simulink model "all_pm_0001_0080"  (R2026a)
settings: Solver=FixedStepAuto  StopTime=50  FixedStep=1e-3  EnableMultiTasking=on
settings Model: PacingRate=0.250000  ExtModeTrigDuration=5  Creator=Arun Mistry  LastModifiedBy=harry_31916
settings OptimizationCC: DefaultUnderspecifiedDataType=single
settings HardwareCC: ProdLargestAtomicInteger=Long  ProdLargestAtomicFloat=Double  ProdHWDeviceType=ARM Compatible->ARM Cortex
settings SFSimCC: SimParseCustomCode=off
settings RTWCC: SystemTargetFile=ert.tlc  Toolchain=GNU Tools for ARM Embedded Processors  Description=Embedded Coder
settings ERTTargetCC: DynamicArrayContainerType=coder::array

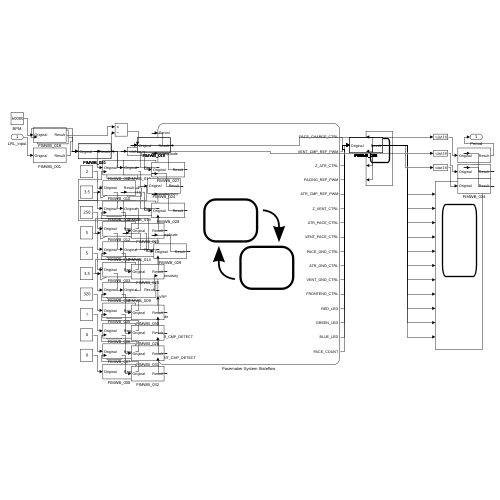
[thumbnail: Simulink's stored preview of the top-level diagram]
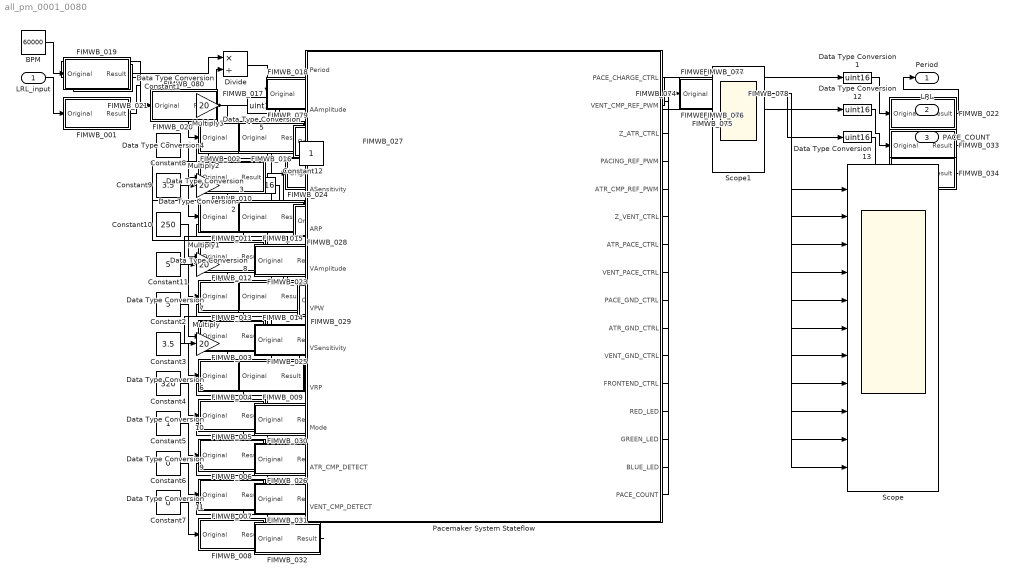
== system all_pm_0001_0080 ==
  LRL_input : Inport  OutDataTypeStr=double
  BPM : Constant  Value=60000
  Constant1 : Constant  Value=5
  Constant10 : Constant  Value=250
  Constant11 : Constant  Value=5
  Constant2 : Constant  Value=5
  Constant3 : Constant  Value=3.5
  Constant4 : Constant  Value=320
  Constant5 : Constant
  Constant6 : Constant  Value=0
  Constant7 : Constant  Value=0
  Constant8 : Constant  Value=2
  Constant9 : Constant  Value=3.5
  Data Type Conversion{,1..8,10,12..13} (12 alike) : DataTypeConversion  OutDataTypeStr=uint16  SaturateOnIntegerOverflow=off  RndMeth=Floor
  Data Type Conversion11 : DataTypeConversion  OutDataTypeStr=boolean  SaturateOnIntegerOverflow=off  RndMeth=Floor
  Data Type Conversion9 : DataTypeConversion  OutDataTypeStr=boolean  SaturateOnIntegerOverflow=off  RndMeth=Floor
  Divide : Product  Inputs=*/
  FIMWB_001 : Subsystem  Tag=fimwb.fault.1
  FIMWB_002 : Subsystem  Tag=fimwb.fault.2
  FIMWB_003 : Subsystem  Tag=fimwb.fault.3
  FIMWB_004 : Subsystem  Tag=fimwb.fault.4
  FIMWB_005 : Subsystem  Tag=fimwb.fault.5
  FIMWB_006 : Subsystem  Tag=fimwb.fault.6
  FIMWB_007 : Subsystem  Tag=fimwb.fault.7
  FIMWB_008 : Subsystem  Tag=fimwb.fault.8
  FIMWB_009 : Subsystem  Tag=fimwb.fault.9
  FIMWB_010 : Subsystem  Tag=fimwb.fault.10
  FIMWB_011 : Subsystem  Tag=fimwb.fault.11
  FIMWB_012 : Subsystem  Tag=fimwb.fault.12
  FIMWB_013 : Subsystem  Tag=fimwb.fault.13
  FIMWB_014 : Subsystem  Tag=fimwb.fault.14
  FIMWB_015 : Subsystem  Tag=fimwb.fault.15
  FIMWB_016 : Subsystem  Tag=fimwb.fault.16
  FIMWB_017 : Subsystem  Tag=fimwb.fault.17
  FIMWB_018 : Subsystem  Tag=fimwb.fault.18
  FIMWB_019 : Subsystem  Tag=fimwb.fault.19
  FIMWB_020 : Subsystem  Tag=fimwb.fault.20
  FIMWB_021 : Subsystem  Tag=fimwb.fault.21
  FIMWB_022 : Subsystem  Tag=fimwb.fault.22
  FIMWB_023 : Subsystem  Tag=fimwb.fault.23
  FIMWB_024 : Subsystem  Tag=fimwb.fault.24
  FIMWB_025 : Subsystem  Tag=fimwb.fault.25
  FIMWB_026 : Subsystem  Tag=fimwb.fault.26
  FIMWB_027 : Subsystem  Tag=fimwb.fault.27
  FIMWB_028 : Subsystem  Tag=fimwb.fault.28
  FIMWB_029 : Subsystem  Tag=fimwb.fault.29
  FIMWB_030 : Subsystem  Tag=fimwb.fault.30
  FIMWB_031 : Subsystem  Tag=fimwb.fault.31
  FIMWB_032 : Subsystem  Tag=fimwb.fault.32
  FIMWB_033 : Subsystem  Tag=fimwb.fault.33
  FIMWB_034 : Subsystem  Tag=fimwb.fault.34
  FIMWB_063 : Subsystem  Tag=fimwb.fault.63
  FIMWB_064 : Subsystem  Tag=fimwb.fault.64
  FIMWB_065 : Subsystem  Tag=fimwb.fault.65
  FIMWB_066 : Subsystem  Tag=fimwb.fault.66
  FIMWB_067 : Subsystem  Tag=fimwb.fault.67
  FIMWB_068 : Subsystem  Tag=fimwb.fault.68
  FIMWB_069 : Subsystem  Tag=fimwb.fault.69
  FIMWB_070 : Subsystem  Tag=fimwb.fault.70
  FIMWB_071 : Subsystem  Tag=fimwb.fault.71
  FIMWB_072 : Subsystem  Tag=fimwb.fault.72
  FIMWB_073 : Subsystem  Tag=fimwb.fault.73
  FIMWB_074 : Subsystem  Tag=fimwb.fault.74
  FIMWB_075 : Subsystem  Tag=fimwb.fault.75
  FIMWB_076 : Subsystem  Tag=fimwb.fault.76
  FIMWB_077 : Subsystem  Tag=fimwb.fault.77
  FIMWB_078 : Subsystem  Tag=fimwb.fault.78
  FIMWB_079 : Subsystem  Tag=fimwb.fault.79
  FIMWB_080 : Subsystem  Tag=fimwb.fault.80
  Multiply{,1..3} (4 alike) : Gain  Gain=20
  Pacemaker System Stateflow : Stateflow chart  TreatAsAtomicUnit=on
  Scope : Scope  NumInputPorts=11
  Scope1 : Scope  NumInputPorts=4
  Period : Outport  OutDataTypeStr=uint16
  LRL : Outport  Port=2  OutDataTypeStr=uint16
  PACE_COUNT : Outport  Port=3
  Constant12 : Constant  IOType=siggen
  wires:
  Divide/1 -> FIMWB_079/1(Original)
  FIMWB_079/1(Result) -> FIMWB_017/1(Original), FIMWB_018/1(Original)
  Data Type Conversion/1 -> FIMWB_080/1(Original)
  FIMWB_080/1(Result) -> FIMWB_020/1(Original), FIMWB_021/1(Original)
  LRL_input/1 -> FIMWB_001/1(Original)
  FIMWB_001/1(Result) -> Data Type Conversion/1
  Constant1/1 -> FIMWB_002/1(Original)
  FIMWB_002/1(Result) -> Multiply3/1
  Constant2/1 -> FIMWB_003/1(Original)
  FIMWB_003/1(Result) -> Data Type Conversion7/1
  Constant3/1 -> FIMWB_004/1(Original)
  FIMWB_004/1(Result) -> Multiply/1
  Constant4/1 -> FIMWB_005/1(Original)
  FIMWB_005/1(Result) -> Data Type Conversion6/1
  Constant5/1 -> FIMWB_006/1(Original)
  FIMWB_006/1(Result) -> Data Type Conversion10/1
  Constant6/1 -> FIMWB_007/1(Original)
  FIMWB_007/1(Result) -> Data Type Conversion9/1
  Constant7/1 -> FIMWB_008/1(Original)
  FIMWB_008/1(Result) -> Data Type Conversion11/1
  Multiply/1 -> FIMWB_009/1(Original)
  FIMWB_009/1(Result) -> Pacemaker System Stateflow/8(VSensitivity)
  Constant8/1 -> FIMWB_010/1(Original)
  FIMWB_010/1(Result) -> Data Type Conversion4/1
  Constant9/1 -> FIMWB_011/1(Original)
  FIMWB_011/1(Result) -> Multiply2/1
  Constant10/1 -> FIMWB_012/1(Original)
  FIMWB_012/1(Result) -> Data Type Conversion2/1
  Constant11/1 -> FIMWB_013/1(Original)
  FIMWB_013/1(Result) -> Multiply1/1
  Multiply1/1 -> FIMWB_014/1(Original)
  FIMWB_014/1(Result) -> Data Type Conversion8/1
  Multiply2/1 -> FIMWB_015/1(Original)
  FIMWB_015/1(Result) -> Data Type Conversion3/1
  Multiply3/1 -> FIMWB_016/1(Original)
  FIMWB_016/1(Result) -> Data Type Conversion5/1
  FIMWB_017/1(Result) -> Data Type Conversion1/1
  FIMWB_018/1(Result) -> Pacemaker System Stateflow/1(Period)
  BPM/1 -> FIMWB_019/1(Original)
  FIMWB_019/1(Result) -> Divide/1
  FIMWB_020/1(Result) -> Divide/2
  FIMWB_021/1(Result) -> Data Type Conversion12/1
  Data Type Conversion1/1 -> FIMWB_022/1(Original)
  FIMWB_022/1(Result) -> Period/1
  Data Type Conversion2/1 -> FIMWB_023/1(Original)
  FIMWB_023/1(Result) -> Pacemaker System Stateflow/5(ARP)
  Data Type Conversion4/1 -> FIMWB_024/1(Original)
  FIMWB_024/1(Result) -> Pacemaker System Stateflow/3(APW)
  Data Type Conversion7/1 -> FIMWB_025/1(Original)
  FIMWB_025/1(Result) -> Pacemaker System Stateflow/7(VPW)
  Data Type Conversion10/1 -> FIMWB_026/1(Original)
  FIMWB_026/1(Result) -> Pacemaker System Stateflow/10(Mode)
  Data Type Conversion5/1 -> FIMWB_027/1(Original)
  FIMWB_027/1(Result) -> Pacemaker System Stateflow/2(AAmplitude)
  Data Type Conversion3/1 -> FIMWB_028/1(Original)
  FIMWB_028/1(Result) -> Pacemaker System Stateflow/4(ASensitivity)
  Data Type Conversion8/1 -> FIMWB_029/1(Original)
  FIMWB_029/1(Result) -> Pacemaker System Stateflow/6(VAmplitude)
  Data Type Conversion6/1 -> FIMWB_030/1(Original)
  FIMWB_030/1(Result) -> Pacemaker System Stateflow/9(VRP)
  Data Type Conversion9/1 -> FIMWB_031/1(Original)
  FIMWB_031/1(Result) -> Pacemaker System Stateflow/11(ATR_CMP_DETECT)
  Data Type Conversion11/1 -> FIMWB_032/1(Original)
  FIMWB_032/1(Result) -> Pacemaker System Stateflow/12(VENT_CMP_DETECT)
  Data Type Conversion12/1 -> FIMWB_033/1(Original)
  FIMWB_033/1(Result) -> LRL/1
  Data Type Conversion13/1 -> FIMWB_034/1(Original)
  FIMWB_034/1(Result) -> PACE_COUNT/1
  Pacemaker System Stateflow/10(ATR_GND_CTRL) -> FIMWB_063/1(Original)
  FIMWB_063/1(Result) -> Scope/6
  Pacemaker System Stateflow/11(VENT_GND_CTRL) -> FIMWB_064/1(Original)
  FIMWB_064/1(Result) -> Scope/7
  Pacemaker System Stateflow/12(FRONTEND_CTRL) -> FIMWB_065/1(Original)
  FIMWB_065/1(Result) -> Scope/8
  Pacemaker System Stateflow/13(RED_LED) -> FIMWB_066/1(Original)
  FIMWB_066/1(Result) -> Scope/9
  Pacemaker System Stateflow/14(GREEN_LED) -> FIMWB_067/1(Original)
  FIMWB_067/1(Result) -> Scope/10
  Pacemaker System Stateflow/15(BLUE_LED) -> FIMWB_068/1(Original)
  FIMWB_068/1(Result) -> Scope/11
  Pacemaker System Stateflow/16(PACE_COUNT) -> FIMWB_069/1(Original)
  FIMWB_069/1(Result) -> Data Type Conversion13/1
  Pacemaker System Stateflow/1(PACE_CHARGE_CTRL) -> FIMWB_070/1(Original)
  FIMWB_070/1(Result) -> Scope1/1
  Pacemaker System Stateflow/2(VENT_CMP_REF_PWM) -> FIMWB_071/1(Original)
  FIMWB_071/1(Result) -> Scope1/2
  Pacemaker System Stateflow/3(Z_ATR_CTRL) -> FIMWB_072/1(Original)
  FIMWB_072/1(Result) -> Scope1/3
  Pacemaker System Stateflow/4(PACING_REF_PWM) -> FIMWB_073/1(Original)
  FIMWB_073/1(Result) -> Scope1/4
  Pacemaker System Stateflow/5(ATR_CMP_REF_PWM) -> FIMWB_074/1(Original)
  FIMWB_074/1(Result) -> Scope/1
  Pacemaker System Stateflow/6(Z_VENT_CTRL) -> FIMWB_075/1(Original)
  FIMWB_075/1(Result) -> Scope/2
  Pacemaker System Stateflow/7(ATR_PACE_CTRL) -> FIMWB_076/1(Original)
  FIMWB_076/1(Result) -> Scope/3
  Pacemaker System Stateflow/8(VENT_PACE_CTRL) -> FIMWB_077/1(Original)
  FIMWB_077/1(Result) -> Scope/4
  Pacemaker System Stateflow/9(PACE_GND_CTRL) -> FIMWB_078/1(Original)
  FIMWB_078/1(Result) -> Scope/5

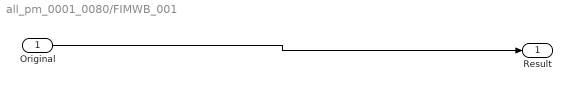
== system all_pm_0001_0080/FIMWB_001 ==
  Original : Inport
  Result : Outport
  wires:
  Original/1 -> Result/1

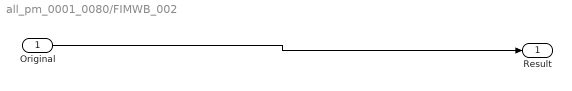
== system all_pm_0001_0080/FIMWB_002 ==
  Original : Inport
  Result : Outport
  wires:
  Original/1 -> Result/1

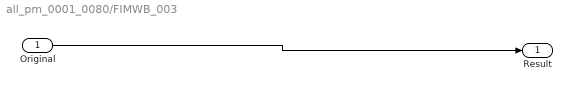
== system all_pm_0001_0080/FIMWB_003 ==
  Original : Inport
  Result : Outport
  wires:
  Original/1 -> Result/1

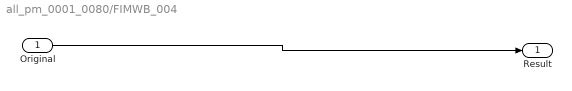
== system all_pm_0001_0080/FIMWB_004 ==
  Original : Inport
  Result : Outport
  wires:
  Original/1 -> Result/1

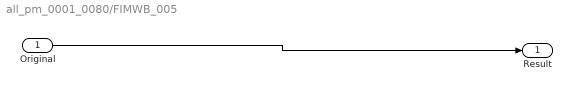
== system all_pm_0001_0080/FIMWB_005 ==
  Original : Inport
  Result : Outport
  wires:
  Original/1 -> Result/1

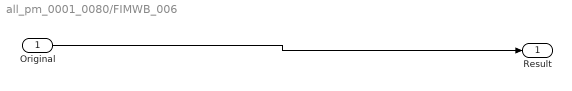
== system all_pm_0001_0080/FIMWB_006 ==
  Original : Inport
  Result : Outport
  wires:
  Original/1 -> Result/1

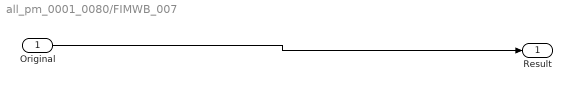
== system all_pm_0001_0080/FIMWB_007 ==
  Original : Inport
  Result : Outport
  wires:
  Original/1 -> Result/1

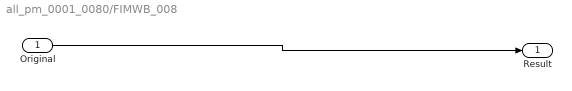
== system all_pm_0001_0080/FIMWB_008 ==
  Original : Inport
  Result : Outport
  wires:
  Original/1 -> Result/1

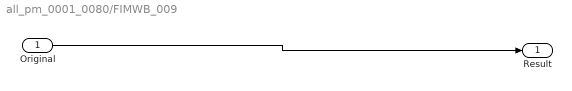
== system all_pm_0001_0080/FIMWB_009 ==
  Original : Inport
  Result : Outport
  wires:
  Original/1 -> Result/1

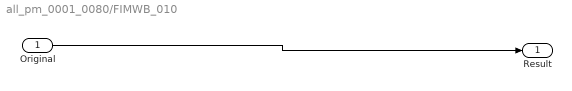
== system all_pm_0001_0080/FIMWB_010 ==
  Original : Inport
  Result : Outport
  wires:
  Original/1 -> Result/1

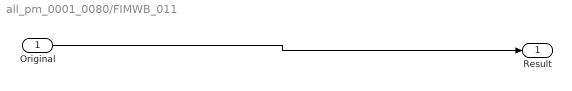
== system all_pm_0001_0080/FIMWB_011 ==
  Original : Inport
  Result : Outport
  wires:
  Original/1 -> Result/1

== system all_pm_0001_0080/FIMWB_012 ==
  Original : Inport
  Result : Outport
  wires:
  Original/1 -> Result/1

== system all_pm_0001_0080/FIMWB_013 ==
  Original : Inport
  Result : Outport
  wires:
  Original/1 -> Result/1

== system all_pm_0001_0080/FIMWB_014 ==
  Original : Inport
  Result : Outport
  wires:
  Original/1 -> Result/1

== system all_pm_0001_0080/FIMWB_015 ==
  Original : Inport
  Result : Outport
  wires:
  Original/1 -> Result/1

== system all_pm_0001_0080/FIMWB_016 ==
  Original : Inport
  Result : Outport
  wires:
  Original/1 -> Result/1

== system all_pm_0001_0080/FIMWB_017 ==
  Original : Inport
  Result : Outport
  wires:
  Original/1 -> Result/1

== system all_pm_0001_0080/FIMWB_018 ==
  Original : Inport
  Result : Outport
  wires:
  Original/1 -> Result/1

== system all_pm_0001_0080/FIMWB_019 ==
  Original : Inport
  Result : Outport
  wires:
  Original/1 -> Result/1

== system all_pm_0001_0080/FIMWB_020 ==
  Original : Inport
  Result : Outport
  wires:
  Original/1 -> Result/1

== system all_pm_0001_0080/FIMWB_021 ==
  Original : Inport
  Result : Outport
  wires:
  Original/1 -> Result/1

== system all_pm_0001_0080/FIMWB_022 ==
  Original : Inport
  Result : Outport
  wires:
  Original/1 -> Result/1

== system all_pm_0001_0080/FIMWB_023 ==
  Original : Inport
  Result : Outport
  wires:
  Original/1 -> Result/1

== system all_pm_0001_0080/FIMWB_024 ==
  Original : Inport
  Result : Outport
  wires:
  Original/1 -> Result/1

== system all_pm_0001_0080/FIMWB_025 ==
  Original : Inport
  Result : Outport
  wires:
  Original/1 -> Result/1

== system all_pm_0001_0080/FIMWB_026 ==
  Original : Inport
  Result : Outport
  wires:
  Original/1 -> Result/1

== system all_pm_0001_0080/FIMWB_027 ==
  Original : Inport
  Result : Outport
  wires:
  Original/1 -> Result/1

== system all_pm_0001_0080/FIMWB_028 ==
  Original : Inport
  Result : Outport
  wires:
  Original/1 -> Result/1

== system all_pm_0001_0080/FIMWB_029 ==
  Original : Inport
  Result : Outport
  wires:
  Original/1 -> Result/1

== system all_pm_0001_0080/FIMWB_030 ==
  Original : Inport
  Result : Outport
  wires:
  Original/1 -> Result/1

== system all_pm_0001_0080/FIMWB_031 ==
  Original : Inport
  Result : Outport
  wires:
  Original/1 -> Result/1

== system all_pm_0001_0080/FIMWB_032 ==
  Original : Inport
  Result : Outport
  wires:
  Original/1 -> Result/1

== system all_pm_0001_0080/FIMWB_033 ==
  Original : Inport
  Result : Outport
  wires:
  Original/1 -> Result/1

== system all_pm_0001_0080/FIMWB_034 ==
  Original : Inport
  Result : Outport
  wires:
  Original/1 -> Result/1

== system all_pm_0001_0080/FIMWB_063 ==
  Original : Inport
  Result : Outport
  wires:
  Original/1 -> Result/1

== system all_pm_0001_0080/FIMWB_064 ==
  Original : Inport
  Result : Outport
  wires:
  Original/1 -> Result/1

== system all_pm_0001_0080/FIMWB_065 ==
  Original : Inport
  Result : Outport
  wires:
  Original/1 -> Result/1

== system all_pm_0001_0080/FIMWB_066 ==
  Original : Inport
  Result : Outport
  wires:
  Original/1 -> Result/1

== system all_pm_0001_0080/FIMWB_067 ==
  Original : Inport
  Result : Outport
  wires:
  Original/1 -> Result/1

== system all_pm_0001_0080/FIMWB_068 ==
  Original : Inport
  Result : Outport
  wires:
  Original/1 -> Result/1

== system all_pm_0001_0080/FIMWB_069 ==
  Original : Inport
  Result : Outport
  wires:
  Original/1 -> Result/1

== system all_pm_0001_0080/FIMWB_070 ==
  Original : Inport
  Result : Outport
  wires:
  Original/1 -> Result/1

== system all_pm_0001_0080/FIMWB_071 ==
  Original : Inport
  Result : Outport
  wires:
  Original/1 -> Result/1

== system all_pm_0001_0080/FIMWB_072 ==
  Original : Inport
  Result : Outport
  wires:
  Original/1 -> Result/1

== system all_pm_0001_0080/FIMWB_073 ==
  Original : Inport
  Result : Outport
  wires:
  Original/1 -> Result/1

== system all_pm_0001_0080/FIMWB_074 ==
  Original : Inport
  Result : Outport
  wires:
  Original/1 -> Result/1

== system all_pm_0001_0080/FIMWB_075 ==
  Original : Inport
  Result : Outport
  wires:
  Original/1 -> Result/1

== system all_pm_0001_0080/FIMWB_076 ==
  Original : Inport
  Result : Outport
  wires:
  Original/1 -> Result/1

== system all_pm_0001_0080/FIMWB_077 ==
  Original : Inport
  Result : Outport
  wires:
  Original/1 -> Result/1

== system all_pm_0001_0080/FIMWB_078 ==
  Original : Inport
  Result : Outport
  wires:
  Original/1 -> Result/1

== system all_pm_0001_0080/FIMWB_079 ==
  Original : Inport
  Result : Outport
  wires:
  Original/1 -> Result/1

== system all_pm_0001_0080/FIMWB_080 ==
  Original : Inport
  Result : Outport
  wires:
  Original/1 -> Result/1

== system all_pm_0001_0080/Pacemaker System Stateflow/FIMWB_035 ==
  Original : Inport
  Result : Outport
  wires:
  Original/1 -> Result/1

== system all_pm_0001_0080/Pacemaker System Stateflow/FIMWB_036 ==
  Original : Inport
  Result : Outport
  wires:
  Original/1 -> Result/1

== system all_pm_0001_0080/Pacemaker System Stateflow/FIMWB_037 ==
  Original : Inport
  Result : Outport
  wires:
  Original/1 -> Result/1

== system all_pm_0001_0080/Pacemaker System Stateflow/FIMWB_038 ==
  Original : Inport
  Result : Outport
  wires:
  Original/1 -> Result/1

== system all_pm_0001_0080/Pacemaker System Stateflow/FIMWB_039 ==
  Original : Inport
  Result : Outport
  wires:
  Original/1 -> Result/1

== system all_pm_0001_0080/Pacemaker System Stateflow/FIMWB_040 ==
  Original : Inport
  Result : Outport
  wires:
  Original/1 -> Result/1

== system all_pm_0001_0080/Pacemaker System Stateflow/FIMWB_041 ==
  Original : Inport
  Result : Outport
  wires:
  Original/1 -> Result/1

== system all_pm_0001_0080/Pacemaker System Stateflow/FIMWB_042 ==
  Original : Inport
  Result : Outport
  wires:
  Original/1 -> Result/1

== system all_pm_0001_0080/Pacemaker System Stateflow/FIMWB_043 ==
  Original : Inport
  Result : Outport
  wires:
  Original/1 -> Result/1

== system all_pm_0001_0080/Pacemaker System Stateflow/FIMWB_044 ==
  Original : Inport
  Result : Outport
  wires:
  Original/1 -> Result/1

== system all_pm_0001_0080/Pacemaker System Stateflow/FIMWB_045 ==
  Original : Inport
  Result : Outport
  wires:
  Original/1 -> Result/1

== system all_pm_0001_0080/Pacemaker System Stateflow/FIMWB_046 ==
  Original : Inport
  Result : Outport
  wires:
  Original/1 -> Result/1

== system all_pm_0001_0080/Pacemaker System Stateflow/FIMWB_047 ==
  Original : Inport
  Result : Outport
  wires:
  Original/1 -> Result/1

== system all_pm_0001_0080/Pacemaker System Stateflow/FIMWB_048 ==
  Original : Inport
  Result : Outport
  wires:
  Original/1 -> Result/1

== system all_pm_0001_0080/Pacemaker System Stateflow/FIMWB_049 ==
  Original : Inport
  Result : Outport
  wires:
  Original/1 -> Result/1

== system all_pm_0001_0080/Pacemaker System Stateflow/FIMWB_050 ==
  Original : Inport
  Result : Outport
  wires:
  Original/1 -> Result/1

== system all_pm_0001_0080/Pacemaker System Stateflow/FIMWB_051 ==
  Original : Inport
  Result : Outport
  wires:
  Original/1 -> Result/1

== system all_pm_0001_0080/Pacemaker System Stateflow/FIMWB_052 ==
  Original : Inport
  Result : Outport
  wires:
  Original/1 -> Result/1

== system all_pm_0001_0080/Pacemaker System Stateflow/FIMWB_053 ==
  Original : Inport
  Result : Outport
  wires:
  Original/1 -> Result/1

== system all_pm_0001_0080/Pacemaker System Stateflow/FIMWB_054 ==
  Original : Inport
  Result : Outport
  wires:
  Original/1 -> Result/1

== system all_pm_0001_0080/Pacemaker System Stateflow/FIMWB_055 ==
  Original : Inport
  Result : Outport
  wires:
  Original/1 -> Result/1

== system all_pm_0001_0080/Pacemaker System Stateflow/FIMWB_056 ==
  Original : Inport
  Result : Outport
  wires:
  Original/1 -> Result/1

== system all_pm_0001_0080/Pacemaker System Stateflow/FIMWB_057 ==
  Original : Inport
  Result : Outport
  wires:
  Original/1 -> Result/1

== system all_pm_0001_0080/Pacemaker System Stateflow/FIMWB_058 ==
  Original : Inport
  Result : Outport
  wires:
  Original/1 -> Result/1

== system all_pm_0001_0080/Pacemaker System Stateflow/FIMWB_059 ==
  Original : Inport
  Result : Outport
  wires:
  Original/1 -> Result/1

== system all_pm_0001_0080/Pacemaker System Stateflow/FIMWB_060 ==
  Original : Inport
  Result : Outport
  wires:
  Original/1 -> Result/1

== system all_pm_0001_0080/Pacemaker System Stateflow/FIMWB_061 ==
  Original : Inport
  Result : Outport
  wires:
  Original/1 -> Result/1

== system all_pm_0001_0080/Pacemaker System Stateflow/FIMWB_062 ==
  Original : Inport
  Result : Outport
  wires:
  Original/1 -> Result/1

== stateflow chart all_pm_0001_0080/Pacemaker System Stateflow ==
  state AOO
    entry: % Initialize pin assigments that do not change during the states
    VENT_PACE_CTRL = 0; VENT_GND_CTRL = 0; PACE_GND_CTRL = 1;
    Z_VENT_CTRL = 0; Z_ATR_CTRL = 0;
    PACING_REF_PWM = AAmplitude; PACE_COUNT = 0;
    state PACE_ATR
      entry:
      % STOP CHARGING C22
      PACE_CHARGE_CTRL = 0;
      % DISCHARGE C22 THROUGH ATR
      ATR_GND_CTRL = 0;
      ATR_PACE_CTRL = 1;
      % PULSING INDICATOR
      BLUE_LED = 1;
      PACE_COUNT = PACE_COUNT + 1;
    state CHARGE_CAPACITOR
      entry:
      % DISCONNECT ATRIAL PACING
      ATR_PACE_CTRL = 0;
      % DISCONNECT C21 FROM GND (allow charge buildup)
      ATR_GND_CTRL = 1;
      % CHARGING C22
      PACE_CHARGE_CTRL = 1;
      % DISABLE PULSING INDICATOR
      BLUE_LED = 0;
    (default) -> AOO.CHARGE_CAPACITOR
    AOO.PACE_ATR -> AOO.CHARGE_CAPACITOR : after(APW,msec)
    AOO.CHARGE_CAPACITOR -> AOO.PACE_ATR : after(Period - 70*APW,msec)
  state MODE_ROUTER
    entry: % Reset these pins when swithching between states
    FRONTEND_CTRL = 1;
    ATR_PACE_CTRL = 0;
    ATR_GND_CTRL = 0;
    VENT_GND_CTRL = 0;
    VENT_PACE_CTRL = 0;
    Z_ATR_CTRL = 0;
    Z_VENT_CTRL = 0;
    GREEN_LED = 0;
    RED_LED = 0;
    BLUE_LED = 0;
  state VOO
    entry: % Initialize pin assigments that do not change during the states
    ATR_PACE_CTRL = 0; ATR_GND_CTRL = 0; PACE_GND_CTRL = 1;
    Z_ATR_CTRL = 0; Z_VENT_CTRL = 0; PACING_REF_PWM = VAmplitude;
    state PACE_VENT
      entry:
      % STOP CHARGING C22
      PACE_CHARGE_CTRL = 0;
      % DISCHARGE C22 THROUGH VENT
      VENT_GND_CTRL = 0;
      VENT_PACE_CTRL = 1;
      % PULSING INDICATOR
      BLUE_LED = 1;
    state CHARGE_CAPACITOR
      entry:
      % DISCONNECT VENT PACING
      VENT_PACE_CTRL = 0;
      % DISCONNECT C21 FROM GND (allow charge to buildup)
      VENT_GND_CTRL = 1;
      % CHARGING C22
      PACE_CHARGE_CTRL = 1;
      % DISABLE PULSING INDICATOR
      BLUE_LED = 0;
    (default) -> VOO.CHARGE_CAPACITOR
    VOO.PACE_VENT -> VOO.CHARGE_CAPACITOR : after(VPW,msec)
    VOO.CHARGE_CAPACITOR -> VOO.PACE_VENT : after(Period-VPW,msec)
  state AAI
    % Initialize pin assignments that do not change during the states
    entry: VENT_PACE_CTRL = 0; VENT_GND_CTRL = 0; PACE_GND_CTRL = 1;
    Z_VENT_CTRL = 0; Z_ATR_CTRL = 0; FRONTEND_CTRL = 1;
    PACING_REF_PWM = AAmplitude; ATR_CMP_REF_PWM=ASensitivity;
    state PACE_ATR
      entry:
      % STOP CHARGING C22
      PACE_CHARGE_CTRL = 0;
      % DISCHARGE C22 THROUGH ATR
      ATR_PACE_CTRL = 1;
      ATR_GND_CTRL = 0;
      % PULSING INDICATOR
      BLUE_LED = 1;
    state C22_CHARGE
      entry:
      % DISCONNECT VENT PACING
      ATR_PACE_CTRL = 0;
      % DISCONNECT C21 FROM GND (allow charge to buildup)
      ATR_GND_CTRL = 1;
      % CHARGING C22
      PACE_CHARGE_CTRL = 1;
    state REFRACTORY_STATE
      % DISABLE PULSING INDICATORS
      entry: BLUE_LED = 0; PACE_CHARGE_CTRL = 1;
      ATR_PACE_CTRL = 0;  ATR_GND_CTRL = 1;
      % DISABLE INHIBIT INIDCATOR ON EXIT
      exit: GREEN_LED = 0;
    (default) -> C22_CHARGE
    C22_CHARGE -> AAI.PACE_ATR [order 2] : after(Period - ARP, msec)
    C22_CHARGE -> REFRACTORY_STATE [order 1] : [ATR_CMP_DETECT]
        | {GREEN_LED = 1}
    REFRACTORY_STATE -> C22_CHARGE : after(ARP, msec)
    AAI.PACE_ATR -> REFRACTORY_STATE : after(APW, msec)
  state VVI
    % Initialize pin assignments that do not change during the states
    entry: ATR_PACE_CTRL = 0; ATR_GND_CTRL = 0; PACE_GND_CTRL = 1;
    Z_VENT_CTRL = 0; Z_ATR_CTRL = 0; FRONTEND_CTRL = 1;
    PACING_REF_PWM = VAmplitude; VENT_CMP_REF_PWM = VSensitivity;
    state PACE_VENT
      entry:
      % STOP CHARGING C22
      PACE_CHARGE_CTRL = 0;
      % DISCHARGE C22 THROUGH VENT
      VENT_PACE_CTRL = 1;
      VENT_GND_CTRL = 0;
      % PULSING INDICATOR
      BLUE_LED = 1;
    state CHARGE_CAPACITOR
      entry:
      % CHARGING C22
      PACE_CHARGE_CTRL = 1;
      % DISCONNECT VENT PACING
      VENT_PACE_CTRL = 0;
      % DISCONNECT FROM GND
      VENT_GND_CTRL = 1;
    state REFRACTORY
      % DISABLE PULSING INDICATOR
      entry: BLUE_LED = 0; PACE_CHARGE_CTRL = 1;
      VENT_PACE_CTRL = 0;  VENT_GND_CTRL = 1;
      % DISABLE INHIBIT INDICATOR ON EXIT (if on)
      exit: GREEN_LED = 0;
    (default) -> VVI.CHARGE_CAPACITOR
    VVI.CHARGE_CAPACITOR -> VVI.PACE_VENT [order 2] : after(Period - VRP, msec)
    VVI.CHARGE_CAPACITOR -> REFRACTORY [order 1] : [VENT_CMP_DETECT]
        | {GREEN_LED = 1}
    REFRACTORY -> VVI.CHARGE_CAPACITOR : after(VRP, msec)
    VVI.PACE_VENT -> REFRACTORY : after(VPW, msec)
  (default) -> MODE_ROUTER
  MODE_ROUTER -> VOO [order 2] : [Mode==2]
  MODE_ROUTER -> AOO [order 1] : [Mode==1]
  VOO -> MODE_ROUTER : [Mode~=2]
  AOO -> MODE_ROUTER : [Mode~=1]
  MODE_ROUTER -> AAI [order 3] : [Mode==3]
  MODE_ROUTER -> VVI [order 4] : [Mode==4]
  AAI -> MODE_ROUTER : [Mode~=3]
  VVI -> MODE_ROUTER : [Mode~=4]
  data: Period input double; AAmplitude input uint16; APW input uint16; ASensitivity input uint16; ARP input uint16; VAmplitude input uint16; VPW input uint16; VSensitivity input double; VRP input uint16; PACE_CHARGE_CTRL output double; VENT_CMP_REF_PWM output double; Z_ATR_CTRL output double; PACING_REF_PWM output uint16; ATR_CMP_REF_PWM output uint16; Z_VENT_CTRL output uint16; ATR_PACE_CTRL output uint16; VENT_PACE_CTRL output uint16; PACE_GND_CTRL output uint16; ATR_GND_CTRL output uint16; VENT_GND_CTRL output uint16; Mode input uint16; FRONTEND_CTRL output uint16; RED_LED output uint16; GREEN_LED output uint16; BLUE_LED output uint16; ATR_CMP_DETECT input boolean; VENT_CMP_DETECT input boolean; PACE_COUNT output
